simulink model "Model_LQR_Real_Kalman"  (R2025a)
settings: Solver=ode4  StartTime=0.0  StopTime=inf  FixedStep=0.0001  RelTol=1e-3
InitFcn:
  | addpath('functions');
model workspace: external: MATLAB File D:\OneDrive - University of Bristol\2025-2026\grp-major_project - General\LQR\LQR_Kalman_Filter\init_LQR_Kalman.m (data not in the file)
values from neighbouring files (symbols this model uses):
  Ad = sys_d.A    [init_LQR_Kalman.m]
  Bd = sys_d.B    [init_LQR_Kalman.m]
  c_omega = (N_gear^2 * Kt * Ke) / R_motor    (= 0.00492477886361)    [init_LQR_Kalman.m]
  c_V = (N_gear * Kt) / R_motor    (= 0.0277237642805)    [init_LQR_Kalman.m]
  Cd = sys_d.C    [init_LQR_Kalman.m]
  fric_1 = [f_v_1, f_c_1, k_fc_1]    [init_LQR_Kalman.m]
  fric_arm = [f_v_arm, f_c_arm, k_fc_arm]    [init_LQR_Kalman.m]
  I_1 = in2(:,4)    [furuta_single_A_B_matrices.m]    (also in furuta_single_state_derivative.m = in4(:,4); init_LQR_Kalman.m = 0.00011)
  I_arm = in2(:,2)    [furuta_single_A_B_matrices.m]    (also in furuta_single_state_derivative.m = in4(:,2); init_LQR_Kalman.m = 0.000739)
  init_S = [0; 0; 0.1; 0]    [init_LQR_Kalman.m]
  K_new = lqr(A_new, B_new, Q, R)    [init_LQR_Kalman.m]
  L = dlqr(Ad', Cd', Q_obs, R_obs)'    [init_LQR_Kalman.m]
  L_1 = 0.14    [init_LQR_Kalman.m]    (also in playback_animation_single.m = out.plotData.L_1.Data(1))
  L_arm = in2(:,1)    [furuta_single_A_B_matrices.m]    (also in furuta_single_state_derivative.m = in4(:,1); init_LQR_Kalman.m = 0.1475; playback_animation_single.m = out.plotData.L_arm.Data(1))
  lcom_1 = in2(:,3)    [furuta_single_A_B_matrices.m]    (also in furuta_single_state_derivative.m = in4(:,3); init_LQR_Kalman.m = 0.051; playback_animation_single.m = out.plotData.lcom_1.Data(1))
  m_1 = in2(:,5)    [furuta_single_A_B_matrices.m]    (also in furuta_single_state_derivative.m = in4(:,5); init_LQR_Kalman.m = 0.054)
settings Model: Creator=Esther  LastModifiedBy=Hankin

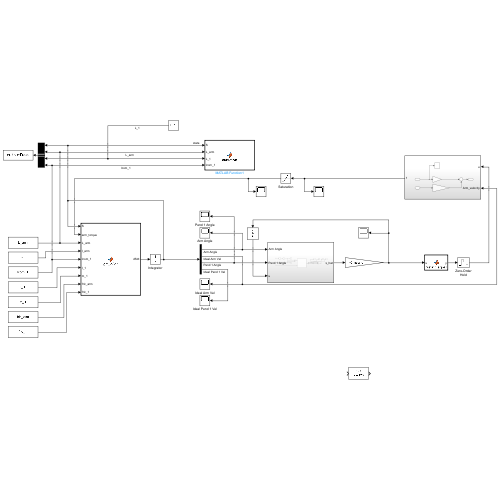
[thumbnail: Simulink's stored preview of the top-level diagram]
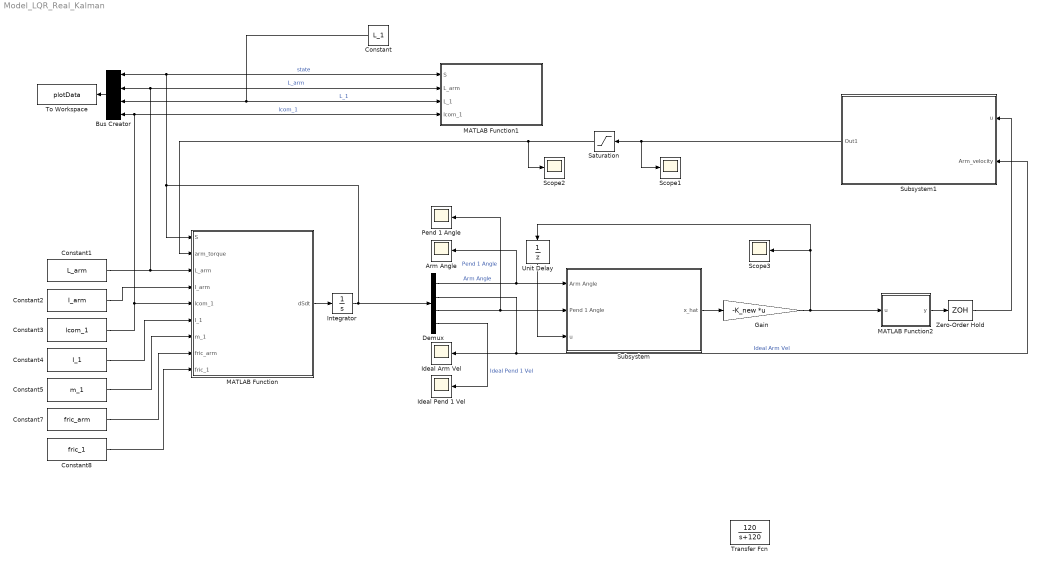
== system Model_LQR_Real_Kalman ==
  Arm Angle : Scope
      settings: ActiveDisplayYMinimum=-0.811685996558267  ActiveDisplayYMaximum=0.70118337402305708
  Bus Creator : BusCreator  Inputs=4
  Constant : Constant  Value=L_1
  Constant1 : Constant  Value=L_arm
  Constant2 : Constant  Value=I_arm
  Constant3 : Constant  Value=lcom_1
  Constant4 : Constant  Value=I_1
  Constant5 : Constant  Value=m_1
  Constant7 : Constant  Value=fric_arm  VectorParams1D=off
  Constant8 : Constant  Value=fric_1  VectorParams1D=off
  Demux : Demux
  Gain : Gain  Gain=-K_new  Multiplication=Matrix(K*u)
  Ideal Arm Vel : Scope
      settings: ActiveDisplayYMinimum=-4.7077852760897549  ActiveDisplayYMaximum=6.144318595660974  DataLoggingVariableName=ScopeData2
  Ideal Pend 1 Vel : Scope
      settings: ActiveDisplayYMinimum=-10.624036988085091  ActiveDisplayYMaximum=10.473809636476057  DataLoggingVariableName=ScopeData4
  Integrator : Integrator  InitialCondition=init_S
  MATLAB Function : MATLAB Function  TreatAsAtomicUnit=on
  MATLAB Function1 : MATLAB Function  TreatAsAtomicUnit=on
  MATLAB Function2 : MATLAB Function  TreatAsAtomicUnit=on
  Pend 1 Angle : Scope
      settings: ActiveDisplayYMinimum=-0.217846735574926  ActiveDisplayYMaximum=0.22165447877793662  DataLoggingVariableName=ScopeData3
  Saturation : Saturate  UpperLimit=0.088  LowerLimit=-0.088  LinearizeAsGain=off
  Scope1 : Scope
      settings: ActiveDisplayYMinimum=-74.7064269652742  ActiveDisplayYMaximum=187.94962601067687  DataLoggingVariableName=ScopeData9
  Scope2 : Scope
      settings: ActiveDisplayYMinimum=-0.10999999999999999  ActiveDisplayYMaximum=0.10999999999999999  DataLoggingVariableName=ScopeData10
  Scope3 : Scope
      settings: ActiveDisplayYMinimum=-74.7064269652742  ActiveDisplayYMaximum=187.94962601067687  DataLoggingVariableName=ScopeData13
  Subsystem : Subsystem
  Subsystem1 : Subsystem
  To Workspace : ToWorkspace  VariableName=plotData  SaveFormat=Timeseries  SampleTime=-1
  Transfer Fcn : TransferFcn  Numerator=[120]  Denominator=[1 120]
  Unit Delay : UnitDelay  SampleTime=-1  HasFrameUpgradeWarning=on
  Zero-Order Hold : ZeroOrderHold  SampleTime=0.001
  wires:
  Constant1/1 -> Bus Creator/2, MATLAB Function1/2(L_arm), MATLAB Function/3(L_arm)  "L_arm"
  Constant2/1 -> MATLAB Function/4(I_arm)
  Constant3/1 -> Bus Creator/4, MATLAB Function1/4(lcom_1), MATLAB Function/5(lcom_1)  "lcom_1"
  Constant4/1 -> MATLAB Function/6(I_1)
  Constant5/1 -> MATLAB Function/7(m_1)
  Integrator/1 -> MATLAB Function/1(S), Bus Creator/1, MATLAB Function1/1(S), Demux/1  "state"
  Bus Creator/1 -> To Workspace/1
  Constant/1 -> MATLAB Function1/3(L_1), Bus Creator/3  "L_1"
  MATLAB Function/1(dSdt) -> Integrator/1
  Demux/1 -> Arm Angle/1, Subsystem/1(Arm Angle)  "Arm Angle"
  Demux/2 -> Ideal Arm Vel/1, Subsystem1/2(Arm_velocity)  "Ideal Arm Vel"
  Demux/3 -> Pend 1 Angle/1, Subsystem/2(Pend 1 Angle)  "Pend 1 Angle"
  Demux/4 -> Ideal Pend 1 Vel/1  "Ideal Pend 1 Vel"
  Saturation/1 -> MATLAB Function/2(arm_torque), Scope2/1
  Subsystem/1(x_hat) -> Gain/1
  Unit Delay/1 -> Subsystem/3(u)
  Constant7/1 -> MATLAB Function/8(fric_arm)
  Constant8/1 -> MATLAB Function/9(fric_1)
  Subsystem1/1(Out1) -> Saturation/1, Scope1/1
  Gain/1 -> MATLAB Function2/1(u), Scope3/1, Unit Delay/1
  MATLAB Function2/1(y) -> Zero-Order Hold/1
  Zero-Order Hold/1 -> Subsystem1/1(u)

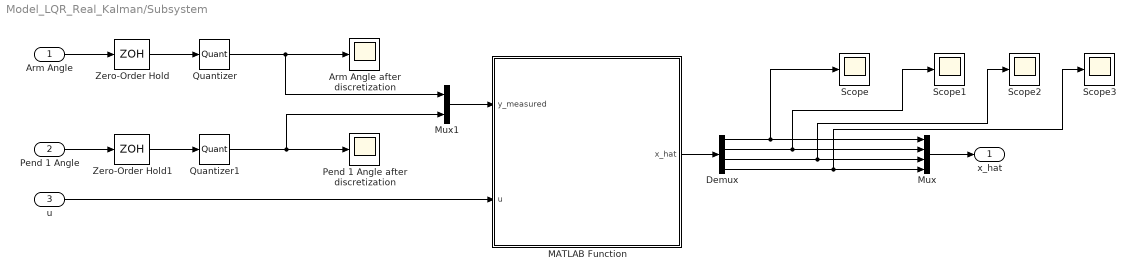
== system Model_LQR_Real_Kalman/Subsystem ==
  Arm Angle : Inport
  Pend 1 Angle : Inport  Port=2
  u : Inport  Port=3
  Arm Angle after discretization : Scope
      settings: ActiveDisplayYMinimum=-0.44610615680975063  ActiveDisplayYMaximum=0.52778756580308528  DataLoggingVariableName=ScopeData5
  Demux : Demux
  MATLAB Function : MATLAB Function  TreatAsAtomicUnit=on
  Mux : Mux
  Mux1 : Mux  Inputs=2
  Pend 1 Angle after discretization : Scope
      settings: ActiveDisplayYMinimum=-1  ActiveDisplayYMaximum=1  DataLoggingVariableName=ScopeData6
  Quantizer : Quantizer  QuantizationInterval=2*pi/408  LinearizeAsGain=off
  Quantizer1 : Quantizer  QuantizationInterval=2*pi/8000  LinearizeAsGain=off
  Scope{,1..3} (4 alike) : Scope
      Scope settings: ActiveDisplayYMinimum=-1  ActiveDisplayYMaximum=1  DataLoggingVariableName=ScopeData7
      Scope1 settings: ActiveDisplayYMinimum=-0.10139192326161425  ActiveDisplayYMaximum=0.096247273484627888  DataLoggingVariableName=ScopeData8
      Scope2 settings: ActiveDisplayYMinimum=-0.062128813184498075  ActiveDisplayYMaximum=0.11874387853705383  DataLoggingVariableName=ScopeData11
      Scope3 settings: ActiveDisplayYMinimum=-0.074206154331659321  ActiveDisplayYMaximum=0.13241901256280292  DataLoggingVariableName=ScopeData12
  Zero-Order Hold : ZeroOrderHold  SampleTime=0.001
  Zero-Order Hold1 : ZeroOrderHold  SampleTime=0.001
  x_hat : Outport
  wires:
  Arm Angle/1 -> Zero-Order Hold/1
  Quantizer1/1 -> Mux1/2, Pend 1 Angle after discretization/1
  Pend 1 Angle/1 -> Zero-Order Hold1/1
  Quantizer/1 -> Arm Angle after discretization/1, Mux1/1
  Mux1/1 -> MATLAB Function/1(y_measured)
  u/1 -> MATLAB Function/2(u)
  MATLAB Function/1(x_hat) -> Demux/1
  Demux/1 -> Scope/1, Mux/1
  Demux/2 -> Mux/2, Scope1/1
  Demux/3 -> Scope2/1, Mux/3
  Mux/1 -> x_hat/1
  Demux/4 -> Scope3/1, Mux/4
  Zero-Order Hold/1 -> Quantizer/1
  Zero-Order Hold1/1 -> Quantizer1/1

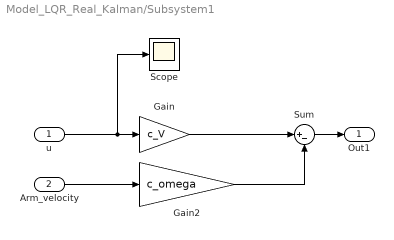
== system Model_LQR_Real_Kalman/Subsystem1 ==
  u : Inport
  Arm_velocity : Inport  Port=2
  Gain : Gain  Gain=c_V
  Gain2 : Gain  Gain=c_omega
  Scope : Scope
      settings: ActiveDisplayYMinimum=-0.7755366956685843  ActiveDisplayYMaximum=0.65253051712373344  DataLoggingVariableName=ScopeData14
  Sum : Sum  Inputs=|+-
  Out1 : Outport
  wires:
  Gain2/1 -> Sum/2
  Gain/1 -> Sum/1
  Arm_velocity/1 -> Gain2/1
  Sum/1 -> Out1/1
  u/1 -> Scope/1, Gain/1

== matlab function Model_LQR_Real_Kalman/MATLAB Function1 ==
  settings: updateMethod=DISCRETE
  data: S input; L_arm input; L_1 input; lcom_1 input
function animation(S, L_arm, L_1, lcom_1)
    update_ratio = 100;
    realtime_animation_single(S, L_arm, L_1, lcom_1, update_ratio);
end

== matlab function Model_LQR_Real_Kalman/MATLAB Function ==
  data: S input size=4; dSdt output size=4; arm_torque input size=1; L_arm input size=1; I_arm input size=1; lcom_1 input size=1; I_1 input size=1; m_1 input size=1; fric_arm input; fric_1 input
function dSdt = get_dSdt(S, arm_torque, L_arm, I_arm, lcom_1, I_1, m_1, fric_arm, fric_1)
    t = 0;
    g = 9.81;
    phys_param = [L_arm, I_arm, lcom_1, I_1, m_1, g];
    dSdt = furuta_single_state_derivative(t, S, arm_torque, phys_param, fric_arm, fric_1);
end

== matlab function Model_LQR_Real_Kalman/Subsystem/MATLAB Function ==
  settings: updateMethod=DISCRETE
  data: y_measured input; u input; x_hat output; Ad parameter; Bd parameter; Cd parameter; L parameter
function x_hat = state_observer(y_measured, u, Ad, Bd, Cd, L)
    % y_measured: 传感器读到的量化角度 [2x1]
    % u: 当前输出的电机力矩 [1x1]
    % x_hat: 观测器输出的估计状态 [4x1]
    
    % 使用 persistent 变量存储上一时刻的状态 (相当于 1/z 延迟模块)
    persistent x_est;
    if isempty(x_est)
        x_est = zeros(4,1); % 初始状态假设为 0
    end
    
    % 1. 当前时刻的输出就是上一时刻预测好的状态
    x_hat = x_est;
    
    % 2. 预测与更新下一时刻的状态 (Luenberger 核心公式)
    % 预测传感器应该读到什么
    y_hat = Cd * x_est; 
    
    % 核心公式：下一时刻状态 = 模型预测 + L * (实际测量 - 模型预测)
    x_est = Ad * x_est + Bd * u + L * (y_measured - y_hat);
end

== matlab function Model_LQR_Real_Kalman/MATLAB Function2 ==
  data: u input; y output
function y = restrict_signal(u)
      % 限制最大值和最小值
      if u > 12
          y = 12;
      elseif u < -12
          y = -12;
      % 限制中心剔除区间 (-0.6, 0.6)
      % 将非负微小信号钳位至正区间下限
      elseif u >= 0 && u < 0.6
          y = 0.6;
      % 将负微小信号钳位至负区间上限
      elseif u < 0 && u > -0.6
          y = -0.6;
      % 信号在正常区间 [-12, -0.6] 或 [0.6, 12] 内，保持原值
      else
          y = u;
      end
  end
